simulink model "native_6dof_validation"  (R2024a)
settings: Solver=ode4  StartTime=0.0  StopTime=2  FixedStep=0.001  RelTol=1e-3
libraries: aerolibprivatev1p5 x1
settings Model: Creator=zz  LastModifiedBy=zz
settings DataIOCC: SaveState=on

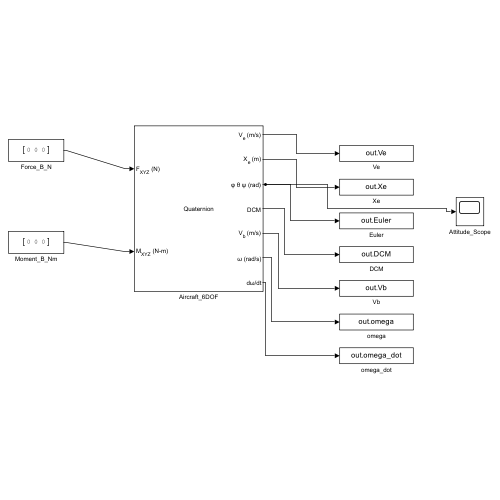
[thumbnail: Simulink's stored preview of the top-level diagram]
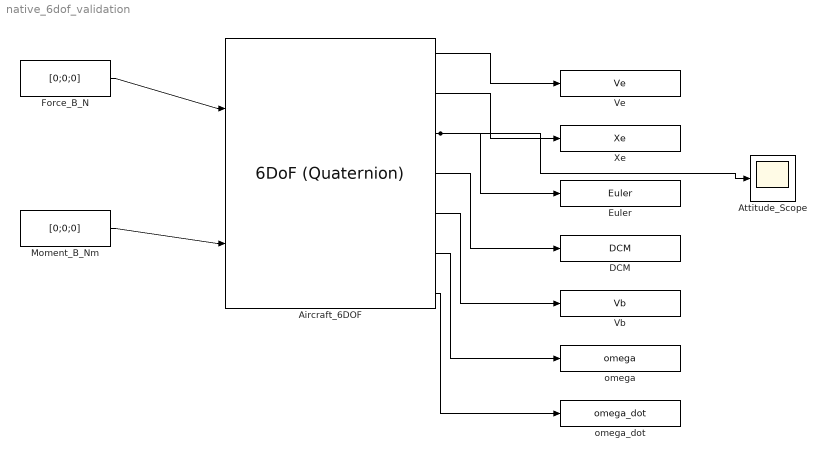
== system native_6dof_validation ==
  Aircraft_6DOF : aerolibprivatev1p5/6DoF (Quaternion)  xme_0=[0 0 0]  Vm_0=[0 0 0]  eul_0=[0 0 0]  pm_0=[0 0 0]  Mass=10  Inertia=diag([2 3 4])  k_quat=1
  Attitude_Scope : Scope
  DCM : ToWorkspace  VariableName=DCM  SaveFormat=Timeseries  SampleTime=-1
  Euler : ToWorkspace  VariableName=Euler  SaveFormat=Timeseries  SampleTime=-1
  Force_B_N : Constant  Value=[0;0;0]
  Moment_B_Nm : Constant  Value=[0;0;0]
  Vb : ToWorkspace  VariableName=Vb  SaveFormat=Timeseries  SampleTime=-1
  Ve : ToWorkspace  VariableName=Ve  SaveFormat=Timeseries  SampleTime=-1
  Xe : ToWorkspace  VariableName=Xe  SaveFormat=Timeseries  SampleTime=-1
  omega : ToWorkspace  VariableName=omega  SaveFormat=Timeseries  SampleTime=-1
  omega_dot : ToWorkspace  VariableName=omega_dot  SaveFormat=Timeseries  SampleTime=-1
  wires:
  Force_B_N/1 -> Aircraft_6DOF/1
  Moment_B_Nm/1 -> Aircraft_6DOF/2
  Aircraft_6DOF/1 -> Ve/1
  Aircraft_6DOF/2 -> Xe/1
  Aircraft_6DOF/3 -> Euler/1, Attitude_Scope/1
  Aircraft_6DOF/4 -> DCM/1
  Aircraft_6DOF/5 -> Vb/1
  Aircraft_6DOF/6 -> omega/1
  Aircraft_6DOF/7 -> omega_dot/1
